simulink model "boost_converter_ANFIS"  (R2026a)
settings: Solver=ode4  StopTime=0.5  FixedStep=1e-05
undefined symbols (not defined in the file): C, L, rL, Rload, Vin, Vref
libraries: fuzblock x1
settings Model: Creator=akash  LastModifiedBy=akash

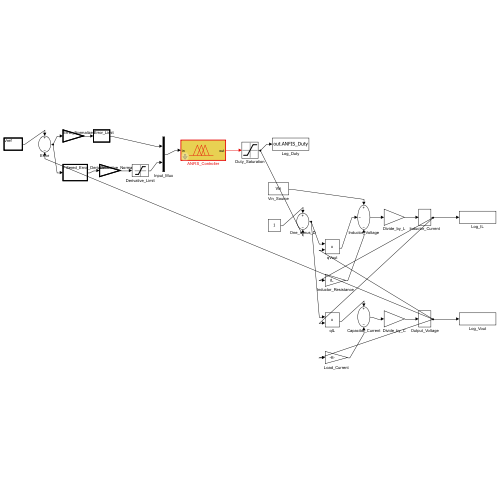
[thumbnail: Simulink's stored preview of the top-level diagram]
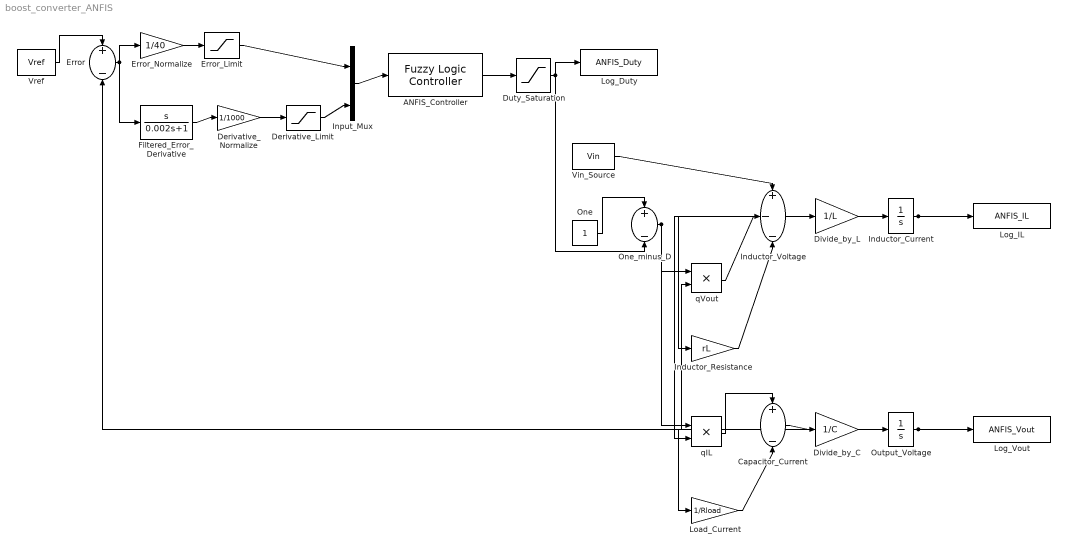
== system boost_converter_ANFIS ==
  ANFIS_Controller : fuzblock/Fuzzy Logic  Controller  FIS=anfisFIS  OutputSampleNumber=101  DataType=double  UseLookupTable=off  NumBreakpoints=10  FuzzifiedInputs=off  RuleFiringStrengths=off  RuleOutputs=off  AggregatedOutputs=off  SimulateUsing=Interpreted execution  OutOfRangeInputValueMessage=warning  NoRuleFiredMessage=warning  EmptyOutputFuzzySetMessage=warning
      settings: LibrarySourceBlock=|
      | fuzblock/Fuzzy Logic
      | Controller
      | with Ruleviewer/Fuzzy Logic
      | Controller
  Capacitor_Current : Sum  Inputs=+-
  Derivative_Limit : Saturate  UpperLimit=1  LowerLimit=-1
  Derivative_Normalize : Gain  Gain=1/1000
  Divide_by_C : Gain  Gain=1/C
  Divide_by_L : Gain  Gain=1/L
  Duty_Saturation : Saturate  UpperLimit=0.65  LowerLimit=0.35
  Error : Sum  Inputs=+-
  Error_Limit : Saturate  UpperLimit=1  LowerLimit=-1
  Error_Normalize : Gain  Gain=1/40
  Filtered_Error_Derivative : TransferFcn  Numerator=[1 0]  Denominator=[0.002 1]
  Inductor_Current : Integrator
  Inductor_Resistance : Gain  Gain=rL
  Inductor_Voltage : Sum  Inputs=+--
  Input_Mux : Mux  Inputs=2
  Load_Current : Gain  Gain=1/Rload
  Log_Duty : ToWorkspace  VariableName=ANFIS_Duty  SaveFormat=Timeseries  SampleTime=-1
  Log_IL : ToWorkspace  VariableName=ANFIS_IL  SaveFormat=Timeseries  SampleTime=-1
  Log_Vout : ToWorkspace  VariableName=ANFIS_Vout  SaveFormat=Timeseries  SampleTime=-1
  One : Constant
  One_minus_D : Sum  Inputs=+-
  Output_Voltage : Integrator
  Vin_Source : Constant  Value=Vin
  Vref : Constant  Value=Vref
  qIL : Product  Inputs=**
  qVout : Product  Inputs=**
  wires:
  Vref/1 -> Error/1
  Output_Voltage/1 -> Error/2, qVout/2, Load_Current/1, Log_Vout/1
  Error/1 -> Error_Normalize/1, Filtered_Error_Derivative/1
  Error_Normalize/1 -> Error_Limit/1
  Filtered_Error_Derivative/1 -> Derivative_Normalize/1
  Derivative_Normalize/1 -> Derivative_Limit/1
  Error_Limit/1 -> Input_Mux/1
  Derivative_Limit/1 -> Input_Mux/2
  Input_Mux/1 -> ANFIS_Controller/1
  ANFIS_Controller/1 -> Duty_Saturation/1
  Duty_Saturation/1 -> Log_Duty/1, One_minus_D/2
  One/1 -> One_minus_D/1
  One_minus_D/1 -> qVout/1, qIL/1
  Inductor_Current/1 -> Inductor_Resistance/1, qIL/2, Log_IL/1
  Vin_Source/1 -> Inductor_Voltage/1
  qVout/1 -> Inductor_Voltage/2
  Inductor_Resistance/1 -> Inductor_Voltage/3
  Inductor_Voltage/1 -> Divide_by_L/1
  Divide_by_L/1 -> Inductor_Current/1
  qIL/1 -> Capacitor_Current/1
  Load_Current/1 -> Capacitor_Current/2
  Capacitor_Current/1 -> Divide_by_C/1
  Divide_by_C/1 -> Output_Voltage/1
